simulink model "ecu_sensaux"  (R2026a)
settings: Solver=FixedStepDiscrete  StopTime=10  FixedStep=0.001  SampleTimeConstraint=STIndependent
Description:
  | Charge-air temperature, pin 79. Source of truth for firmware/gen/ecu_sensaux.
settings Model: Creator=jj1001000  LastModifiedBy=jj1001000
settings OptimizationCC: DefaultUnderspecifiedDataType=single
settings DebuggingCC: ParameterPrecisionLossMsg=none
settings HardwareCC: ProdLargestAtomicInteger=Long  ProdLargestAtomicFloat=Double  ProdHWDeviceType=ARM Compatible->ARM Cortex-M
settings RTWCC: SystemTargetFile=ert.tlc  GenCodeOnly=on  Description=Embedded Coder
settings ERTTargetCC: UtilityFuncGeneration=Shared location  IncludeMdlTerminateFcn=off  CodeInterfacePackaging=Reusable function  SupportNonFinite=off

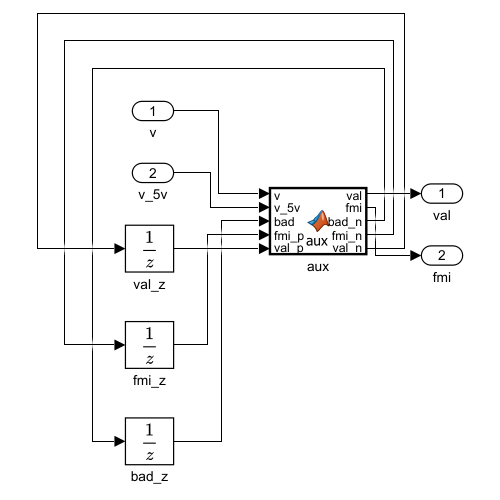
[thumbnail: Simulink's stored preview of the top-level diagram]
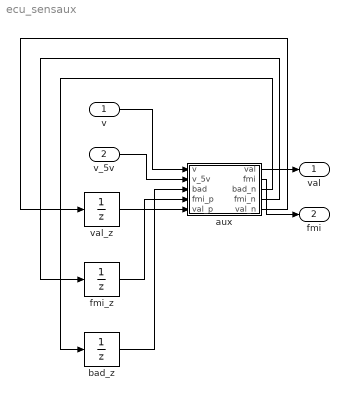
== system ecu_sensaux ==
  v : Inport  OutDataTypeStr=single
  v_5v : Inport  Port=2  OutDataTypeStr=single
  aux : MATLAB Function  TreatAsAtomicUnit=on
  bad_z : UnitDelay  SampleTime=-1
  fmi_z : UnitDelay  SampleTime=-1
  val_z : UnitDelay  InitialCondition=40  SampleTime=-1
  val : Outport  OutDataTypeStr=single
  fmi : Outport  Port=2  OutDataTypeStr=uint8
  wires:
  v/1 -> aux/1(v)
  v_5v/1 -> aux/2(v_5v)
  fmi_z/1 -> aux/4(fmi_p)
  val_z/1 -> aux/5(val_p)
  bad_z/1 -> aux/3(bad)
  aux/1(val) -> val/1
  aux/3(bad_n) -> bad_z/1
  aux/2(fmi) -> fmi/1
  aux/4(fmi_n) -> fmi_z/1
  aux/5(val_n) -> val_z/1

== matlab function ecu_sensaux/aux ==
  data: v input single; val output single; v_5v input single; bad input uint16; fmi_p input uint8; val_p input single; fmi output uint8; bad_n output uint16; fmi_n output uint8; val_n output single
function [val, fmi, bad_n, fmi_n, val_n] = aux(v, v_5v, bad, fmi_p, val_p)
%#codegen
NT = single([-40 -30 -20 -10 0 10 20 30 40 50 60 70 80 90 100 110 120 130 140 150]); NR = single([45313 26114 15462 9397 5896 3792 2500 1707 1175 834 596 436 323 243 187 144 113 89 71 57]);
v5 = v_5v;
if ~(v5 >= single(4.5) && v5 <= single(5.5))
    v5 = single(5);
end
bad_n = bad; fmi_n = fmi_p; val_n = val_p;
vr = v * single(5) / v5;
if ~(vr <= single(4.80000019))
    now = uint8(3);
elseif vr < single(0.100000001)
    now = uint8(4);
else
    now = uint8(0);
end
if (now ~= 0) ~= (fmi_n ~= 0)
    bad_n = bad_n + uint16(1);
    if bad_n >= uint16(100)
        fmi_n = now;
        bad_n = uint16(0);
    end
else
    bad_n = uint16(0);
    if now ~= 0
        fmi_n = now;
    end
end
if fmi_n ~= 0
    val_n = single(40);
elseif now == 0
    r = single(2490) * vr / (single(5) - vr);
    if r < single(260000)
        r = r * single(260000) / (single(260000) - r);
    else
        r = single(1e9);
    end
    if ~(r < NR(1))
        val_n = NT(1);
    elseif r <= NR(20)
        val_n = NT(20);
    else
        k = int32(1);
        while r <= NR(k + 1)
            k = k + int32(1);
        end
        val_n = NT(k) + (NT(k + 1) - NT(k)) * (log(NR(k) / r) / log(NR(k) / NR(k + 1)));
    end
end
val = val_n; fmi = fmi_n;
